simulink model "online_robot_2024b"  (R2024b)
settings: Solver=FixedStepAuto  StartTime=0.0  StopTime=inf  RelTol=1e-3
undefined symbols (not defined in the file): control_par, controller_index, d, D, is_real_robot, k_theta, k_x, k_y, P_INIT_EKF, q_goal_task1, q_goal_task2, q_init, r, R_2, R_5, R_bad, R_good, T_s, Ts, X, Y
libraries: robotlib x6, simulink x5, sharedtransform x1
(part 1 of 2)
settings Model: SimulationMode=accelerator  Creator=dallaliber  LastModifiedBy=HOSAM
settings OptimizationCC: DefaultParameterBehavior=Inlined  EnhancedBackFolding=on  PassReuseOutputArgsAs=Individual arguments  ZeroExternalMemoryAtStartup=off  ZeroInternalMemoryAtStartup=off  MaxStackSize=64  OptimizeBlockOrder=speed  DifferentSizesBufferReuse=on  OptimizationCustomize=off  EfficientTunableParamExpr=on
settings DebuggingCC: ParameterTunabilityLossMsg=error
settings HardwareCC: ProdBitPerPointer=32  ProdBitPerSizeT=32  ProdBitPerPtrDiffT=32  ProdLargestAtomicFloat=None  ProdIntDivRoundTo=Undefined  ProdEndianess=Unspecified  ProdWordSize=32  ProdHWDeviceType=Generic->Unspecified (assume 32-bit Generic)
settings SFSimCC: MATLABDynamicMemAlloc=off
settings RTWCC: Description=Embedded Coder  SystemTargetFile=ert.tlc  HardwareBoard=Robot Operating System (ROS)  TLCOptions="-aInlineSetEventsForThisBaseRateFcn=TLC_FALSE -aSuppressMultiTaskScheduler=TLC_FALSE  -aRateBasedStepFcn=0"  TemplateMakefile=ert_default_tmf  Toolchain=Catkin  TargetLang=C++
settings CodeAppCC: ForceParamTrailComments=on  IgnoreCustomStorageClasses=off  OperatorAnnotations=on  SimulinkDataObjDesc=on  SFDataObjDesc=on  InsertBlockDesc=on
settings ERTTargetCC: DynamicArrayContainerType=coder::array
settings ConfigComp: CovBoundaryAbsTol=1.0e-5

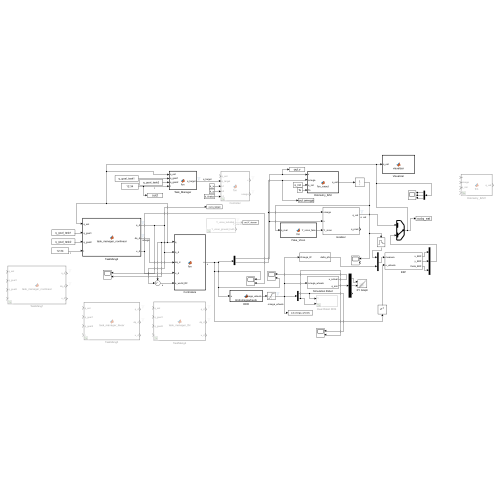
[thumbnail: Simulink's stored preview of the top-level diagram]
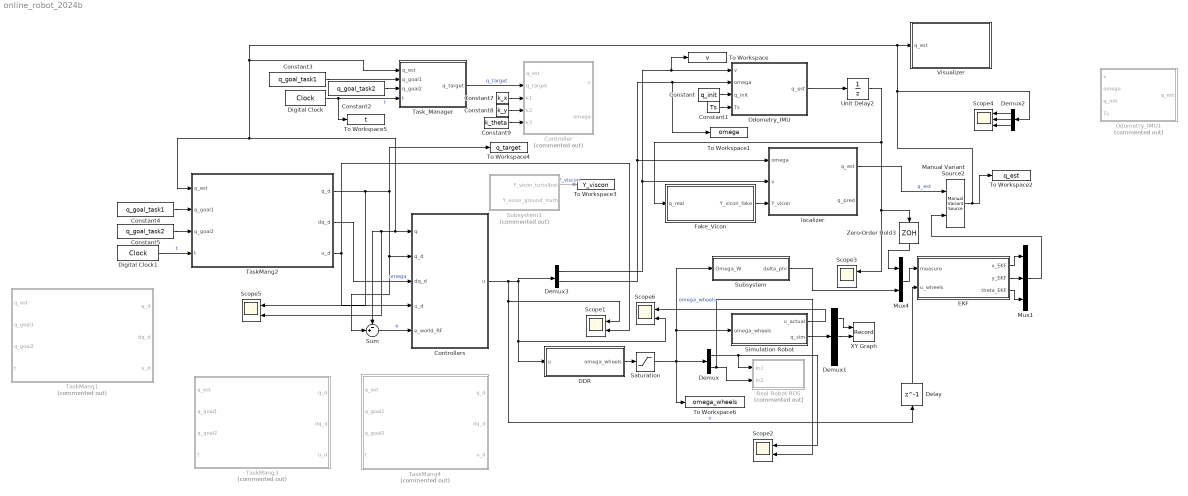
== system online_robot_2024b ==
  Constant : Constant  Value=q_init  SampleTime=Ts
  Constant1 : Constant  Value=Ts  SampleTime=Ts
  Constant2 : Constant  Value=q_goal_task2  SampleTime=Ts
  Constant3 : Constant  Value=q_goal_task1  SampleTime=Ts
  Constant4 : Constant  Value=q_goal_task1  SampleTime=Ts
  Constant5 : Constant  Value=q_goal_task2  SampleTime=Ts
  Constant7 : Constant  Value=k_x  SampleTime=Ts
  Constant8 : Constant  Value=k_y  SampleTime=Ts
  Constant9 : Constant  Value=k_theta  SampleTime=Ts
  Controller : MATLAB Function  Commented=on  TreatAsAtomicUnit=on
  Controllers : MATLAB Function  TreatAsAtomicUnit=on
  DDR : MATLAB Function  TreatAsAtomicUnit=on
  Delay : Delay  DelayLength=1  InitialCondition=[0;0]  SampleTime=Ts
  Demux : Demux  Outputs=2
  Demux1 : Demux  Outputs=3
  Demux2 : Demux  Outputs=3
  Demux3 : Demux  Outputs=2
  Digital Clock : DigitalClock  SampleTime=Ts
  Digital Clock1 : DigitalClock  SampleTime=Ts
  EKF : Subsystem
  Fake_Vicon : MATLAB Function  TreatAsAtomicUnit=on
  Manual Variant Source2 : simulink/Signal Routing/Manual Variant Source  NumChoices=2  LabelModeActiveChoice=V_2
  Mux1 : Mux  Inputs=3
  Mux4 : Mux  Inputs=2
  Odometry_IMU : MATLAB Function  TreatAsAtomicUnit=on
  Odometry_IMU1 : MATLAB Function  Commented=on  TreatAsAtomicUnit=on
  Real Robot ROS : Subsystem  Commented=on
  Saturation : Saturate  UpperLimit=10  LowerLimit=-10
  Scope{1..3,5..6} (5 alike) : Scope  NumInputPorts=2
  Scope4 : Scope  NumInputPorts=3
  Simulation Robot : Subsystem
  Subsystem : Subsystem
  Subsystem1 : Subsystem  Commented=on
  Sum : Sum  Inputs=-+|
  TaskMang1 : MATLAB Function  Commented=on  TreatAsAtomicUnit=on
  TaskMang2 : MATLAB Function  TreatAsAtomicUnit=on
  TaskMang3 : MATLAB Function  Commented=on  TreatAsAtomicUnit=on
  TaskMang4 : MATLAB Function  Commented=on  TreatAsAtomicUnit=on
  Task_Manager : MATLAB Function  TreatAsAtomicUnit=on
  To Workspace : ToWorkspace  VariableName=v  SampleTime=Ts
  To Workspace1 : ToWorkspace  VariableName=omega  SampleTime=Ts
  To Workspace2 : ToWorkspace  VariableName=q_est  SampleTime=Ts
  To Workspace3 : ToWorkspace  VariableName=Y_viscon  SampleTime=Ts
  To Workspace4 : ToWorkspace  VariableName=q_target  SampleTime=Ts
  To Workspace5 : ToWorkspace  VariableName=t  SampleTime=Ts
  To Workspace6 : ToWorkspace  VariableName=omega_wheels  SampleTime=Ts
  Unit Delay2 : UnitDelay  InitialCondition=q_init  SampleTime=Ts  HasFrameUpgradeWarning=on
  Visualizer : MATLAB Function  TreatAsAtomicUnit=on
  XY Graph : Record  FileSettingsInternal="{\"entries\":[{\"content\":{\"excelSettings\":{\"content\":{},\"type\":\"Streamout.ExcelSettings\"},\"parquetSettings\":{\"content\":{},\"type\":\"Streamout.ParquetSettings\"}},\"type\":\"Streamout.FileSettingStorage\",\"uuid\":\"\"}],\"packageUris\":[\"http:\\/\\/schema.mathworks.com\\/mf0\\/streamout_blocks\\/R2020a\"],\"version\":\"1.0\"}"  Layout=[1 1]  SignalsInternal="{\"entries\":[{\"content\":{\"signals\":[{\"content\":{\"blockPath\":[],\"dimensions\":[1],\"domain\":\"\",\"lineColor\":\"#a2142f\",\"plots\":[ 1 ],\"port\":1,\"signalID\":1,\"signalName\":\"Demux1:1\"},\"type\":\"RecordBlkView.Signal\",\"uuid\":\"\"},{\"content\":{\"blockPath\":[],\"dimensions\":[1],\"domain\":\"\",\"lineColor\":\"#139fff\",\"plots\":[ 1 ],\"port\":2,\"signalID\":2,\"signalName\":\"Demux1:2\"},\"type\":\"RecordBlkView.Signal\",\"uuid\":\"\"}]},\"type\":\"RecordBlkView.InputSignals\",\"uuid\":\"\"}],\"packageUris\":[\"http:\\/\\/schema.mathworks.com\\/mf0\\/streamout_blocks\\/R2020a\"],\"version\":\"1.0\"}"  VisualizationBindings="{\"xyplotplugin\":{\"info\":[{\"series\":[{\"bindingParametersList\":[{\"parameter\":\"X-Axis\",\"signalID\":1,\"signalName\":\"Demux1:1\"},{\"parameter\":\"Y-Axis\",\"signalID\":2,\"signalName\":\"Demux1:2\"}],\"seriesID\":0}],\"subplotID\":1}]}}"  CompatibilityTag=XY
  Zero-Order Hold3 : ZeroOrderHold  SampleTime=T_s
  localizer : Subsystem
  wires:
  Constant/1 -> Odometry_IMU/3(q_init)
  Constant1/1 -> Odometry_IMU/4(Ts)
  Constant2/1 -> Task_Manager/3(q_goal2)
  Constant3/1 -> Task_Manager/2(q_goal1)
  Odometry_IMU/1(q_est) -> Unit Delay2/1
  Saturation/1 -> Subsystem/1(Omega_W), Simulation Robot/1(omega_wheels), To Workspace6/1, Demux/1  "omega_wheels"
  DDR/1(omega_wheels) -> Saturation/1
  Demux/1 -> Scope2/1, Real Robot ROS/1(In1)
  Demux/2 -> Scope2/2, Real Robot ROS/2(In2)
  Digital Clock/1 -> To Workspace5/1, Task_Manager/4(t)  "t"
  Subsystem1/1(Y_vicon_turtulbot) -> To Workspace3/1  "Y_viscon"
  Task_Manager/1(q_target) -> Controller/2(q_target)  "q_target"
  Constant7/1 -> Controller/3(k1)
  Constant8/1 -> Controller/4(k2)
  Constant9/1 -> Controller/5(k3)
  Fake_Vicon/1(Y_vicon_fake) -> localizer/3(Y_vicon)
  Unit Delay2/1 -> Zero-Order Hold3/1, Scope3/1, Fake_Vicon/1(q_real)
  Simulation Robot/2(q_sim) -> Demux1/1
  Demux2/3 -> Scope4/3
  Demux2/1 -> Scope4/1
  Demux2/2 -> Scope4/2
  Demux1/1 -> XY Graph/1
  Demux1/2 -> XY Graph/2
  Constant4/1 -> TaskMang2/2(q_goal1)
  Constant5/1 -> TaskMang2/3(q_goal2)
  Digital Clock1/1 -> TaskMang2/4(t)  "t"
  TaskMang2/1(q_d) -> Sum/2, Controllers/2(q_d), To Workspace4/1, Scope5/1
  TaskMang2/2(dq_d) -> Controllers/3(dq_d)  "omega"
  TaskMang2/3(u_d) -> Controllers/4(u_d), Scope1/2
  Sum/1 -> Controllers/5(e_world_RF)  "e"
  Controllers/1(u) -> Delay/1, Scope1/1, Demux3/1, Scope6/2, DDR/1(u)  "u"
  Demux3/1 -> To Workspace/1, Odometry_IMU/1(v), localizer/2(v)
  Demux3/2 -> To Workspace1/1, Odometry_IMU/2(omega), localizer/1(omega)
  EKF/2(y_EKF) -> Mux1/2
  EKF/1(x_EKF) -> Mux1/1
  EKF/3(theta_EKF) -> Mux1/3
  Subsystem/1(delta_phi) -> Mux4/2
  Zero-Order Hold3/1 -> Mux4/1
  Mux4/1 -> EKF/1(measure)
  Manual Variant Source2/1 -> Task_Manager/1(q_est), Controllers/1(q), Scope5/2, Sum/1, TaskMang2/1(q_est), Visualizer/1(q_est), Demux2/1, To Workspace2/1
  localizer/1(q_est) -> Manual Variant Source2/1  "q_est"
  Mux1/1 -> Manual Variant Source2/2
  Simulation Robot/1(u_actual) -> Scope6/1
  Delay/1 -> EKF/2(u_wheels)

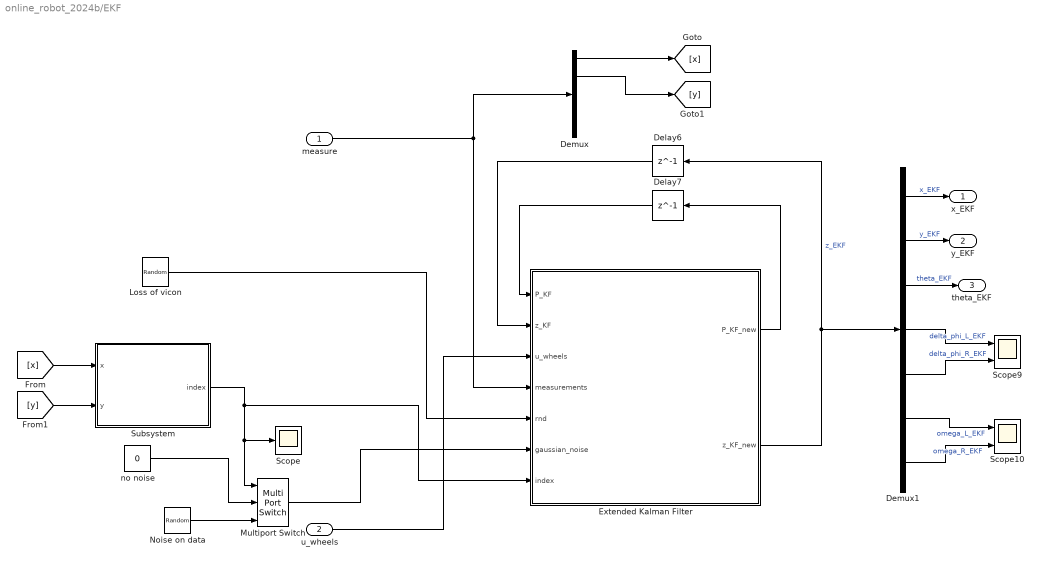
== system online_robot_2024b/EKF ==
  measure : Inport
  u_wheels : Inport  Port=2
  " Loss of vicon" : UniformRandomNumber  Minimum=0  SampleTime=Ts
  Delay6 : Delay  DelayLength=1  InitialCondition=[q_init; 0; 0; 0; 0]  SampleTime=Ts
  Delay7 : Delay  DelayLength=1  InitialCondition=P_INIT_EKF  SampleTime=Ts
  Demux : Demux  Outputs=5
  Demux1 : Demux  Outputs=7
  Extended Kalman Filter : MATLAB Function  TreatAsAtomicUnit=on
  Multiport Switch : MultiPortSwitch  Inputs=2  SaturateOnIntegerOverflow=off  InputSameDT=off
  Noise on data : RandomNumber  Variance=0.02^2  SampleTime=Ts
  Scope : Scope
  Scope10 : Scope  NumInputPorts=2
  Scope9 : Scope  NumInputPorts=2
  Subsystem : Subsystem
  no noise : Constant  Value=0
  x_EKF : Outport
  y_EKF : Outport  Port=2
  theta_EKF : Outport  Port=3
  wires:
  Demux1/6 -> Scope10/1  "omega_L_EKF"
  Demux1/3 -> theta_EKF/1  "theta_EKF"
  Delay6/1 -> Extended Kalman Filter/2(z_KF)
  Delay7/1 -> Extended Kalman Filter/1(P_KF)
  Demux1/5 -> Scope9/2  "delta_phi_R_EKF"
  Demux1/7 -> Scope10/2  "omega_R_EKF"
  Extended Kalman Filter/1(P_KF_new) -> Delay7/1
  Multiport Switch/1 -> Extended Kalman Filter/6(gaussian_noise)
  " Loss of vicon"/1 -> Extended Kalman Filter/5(rnd)
  Demux1/1 -> x_EKF/1  "x_EKF"
  Demux1/4 -> Scope9/1  "delta_phi_L_EKF"
  u_wheels/1 -> Extended Kalman Filter/3(u_wheels)
  Extended Kalman Filter/2(z_KF_new) -> Demux1/1, Delay6/1  "z_EKF"
  measure/1 -> Demux/1, Extended Kalman Filter/4(measurements)
  Demux1/2 -> y_EKF/1  "y_EKF"
  Subsystem/1(index) -> Extended Kalman Filter/7(index), Multiport Switch/1, Scope/1
  [x] -> Subsystem/1(x)
  Noise on data/1 -> Multiport Switch/3
  no noise/1 -> Multiport Switch/2
  [y] -> Subsystem/2(y)
  Demux/1 -> [x]
  Demux/2 -> [y]

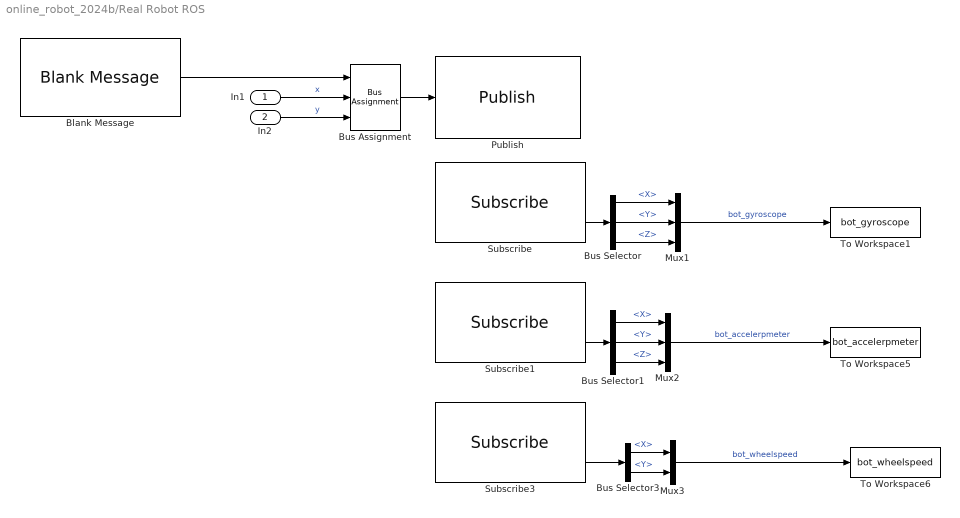
== system online_robot_2024b/Real Robot ROS ==
  In1 : Inport
  In2 : Inport  Port=2
  Blank Message : robotlib/Blank Message  messageClass=Message  entityType=geometry_msgs/Vector3  messageType=geometry_msgs/Vector3  SampleTime=0.04  legacyBusStruct=off
  Bus Assignment : BusAssignment  AssignedSignals=X,Y
  Bus Selector : BusSelector  OutputSignals=X,Y,Z
  Bus Selector1 : BusSelector  OutputSignals=X,Y,Z
  Bus Selector3 : BusSelector  OutputSignals=X,Y
  Mux1 : Mux  Inputs=3
  Mux2 : Mux  Inputs=3
  Mux3 : Mux  Inputs=2
  Publish : robotlib/Publish  topicSource=Select from ROS network  topic=/turtlebot_09/cmd_wheels  messageType=geometry_msgs/Vector3  legacyBusStruct=off  messageQueueLength=1
  Subscribe : robotlib/Subscribe  topicSource=Select from ROS network  topic=/turtlebot_09/gyroscope  messageType=geometry_msgs/Vector3  SampleTime=0.04  legacyBusStruct=off  messageQueueLength=1
  Subscribe1 : robotlib/Subscribe  topicSource=Select from ROS network  topic=/turtlebot_09/accelerometer  messageType=geometry_msgs/Vector3  SampleTime=0.04  legacyBusStruct=off  messageQueueLength=1
  Subscribe3 : robotlib/Subscribe  topicSource=Select from ROS network  topic=/turtlebot_09/wheelSpeeds  messageType=geometry_msgs/Vector3  SampleTime=0.04  legacyBusStruct=off  messageQueueLength=1
  To Workspace1 : ToWorkspace  VariableName=bot_gyroscope  SaveFormat=Timeseries  SampleTime=Ts
  To Workspace5 : ToWorkspace  VariableName=bot_accelerpmeter  SaveFormat=Timeseries  SampleTime=Ts
  To Workspace6 : ToWorkspace  VariableName=bot_wheelspeed  SaveFormat=Timeseries  SampleTime=Ts
  wires:
  Subscribe1/2 -> Bus Selector1/1
  Bus Selector1/1 -> Mux2/1  "<X>"
  Mux2/1 -> To Workspace5/1  "bot_accelerpmeter"
  Bus Assignment/1 -> Publish/1
  Subscribe/2 -> Bus Selector/1
  In2/1 -> Bus Assignment/3  "y"
  Bus Selector/2 -> Mux1/2  "<Y>"
  Bus Selector/1 -> Mux1/1  "<X>"
  Bus Selector3/1 -> Mux3/1  "<X>"
  Bus Selector3/2 -> Mux3/2  "<Y>"
  Bus Selector1/3 -> Mux2/3  "<Z>"
  Bus Selector1/2 -> Mux2/2  "<Y>"
  Mux3/1 -> To Workspace6/1  "bot_wheelspeed"
  Mux1/1 -> To Workspace1/1  "bot_gyroscope"
  Subscribe3/2 -> Bus Selector3/1
  In1/1 -> Bus Assignment/2  "x"
  Blank Message/1 -> Bus Assignment/1
  Bus Selector/3 -> Mux1/3  "<Z>"

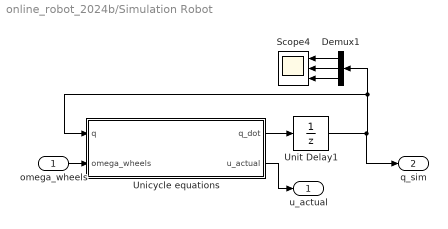
== system online_robot_2024b/Simulation Robot ==
  omega_wheels : Inport
  Demux1 : Demux  Outputs=3
  Scope4 : Scope  NumInputPorts=3
  Unicycle equations : MATLAB Function  TreatAsAtomicUnit=on
  Unit Delay1 : UnitDelay  InitialCondition=q_init  SampleTime=Ts  HasFrameUpgradeWarning=on
  u_actual : Outport
  q_sim : Outport  Port=2
  wires:
  Unicycle equations/1(q_dot) -> Unit Delay1/1
  Demux1/2 -> Scope4/2
  Demux1/1 -> Scope4/1
  Unicycle equations/2(u_actual) -> u_actual/1
  omega_wheels/1 -> Unicycle equations/2(omega_wheels)
  Unit Delay1/1 -> q_sim/1, Unicycle equations/1(q), Demux1/1
  Demux1/3 -> Scope4/3

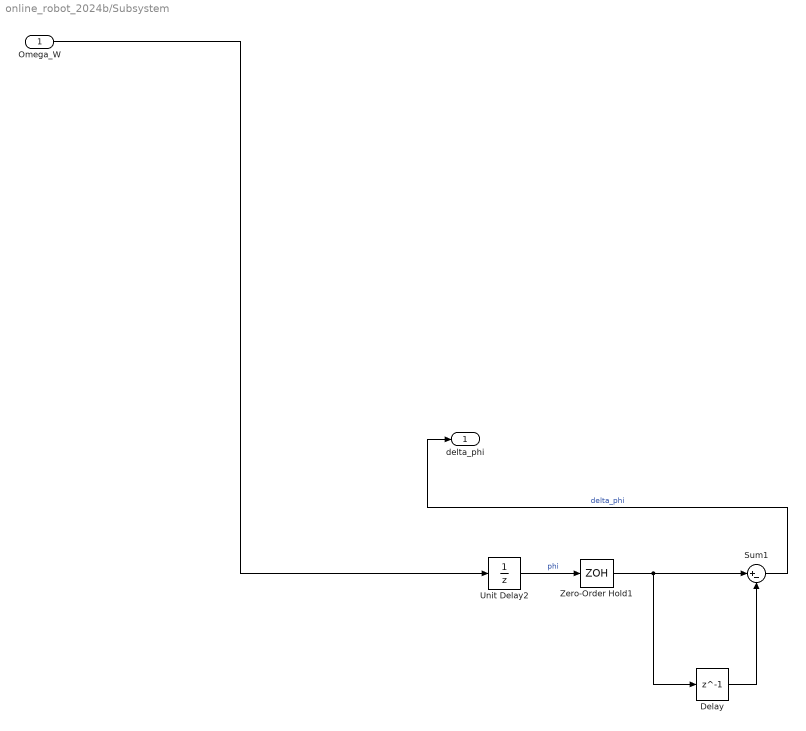
== system online_robot_2024b/Subsystem ==
  Omega_W : Inport
  Delay : Delay  DelayLength=1  InitialCondition=[0;0]  SampleTime=T_s
  Sum1 : Sum  Inputs=|+-
  Unit Delay2 : UnitDelay  InitialCondition=[0;0]  SampleTime=Ts  HasFrameUpgradeWarning=on
  Zero-Order Hold1 : ZeroOrderHold  SampleTime=T_s
  delta_phi : Outport
  wires:
  Sum1/1 -> delta_phi/1  "delta_phi"
  Omega_W/1 -> Unit Delay2/1
  Zero-Order Hold1/1 -> Sum1/1, Delay/1
  Delay/1 -> Sum1/2
  Unit Delay2/1 -> Zero-Order Hold1/1  "phi"

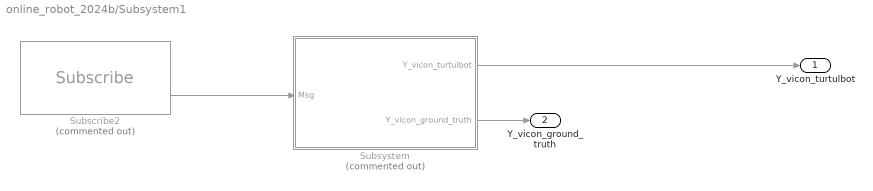
== system online_robot_2024b/Subsystem1 ==
  Subscribe2 : robotlib/Subscribe  Commented=on  topicSource=Select from ROS network  topic=/turtlebot_09/odom  messageType=nav_msgs/Odometry  SampleTime=Ts  legacyBusStruct=off  messageQueueLength=1
      settings: LibrarySourceBlock=roslib/ROS/Subscribe
  Subsystem : Subsystem  Commented=on
  Y_vicon_turtulbot : Outport
  Y_vicon_ground_truth : Outport  Port=2
  wires:
  Subscribe2/2 -> Subsystem/1(Msg)
  Subsystem/2(Y_vicon_ground_truth) -> Y_vicon_ground_truth/1
  Subsystem/1(Y_vicon_turtulbot) -> Y_vicon_turtulbot/1

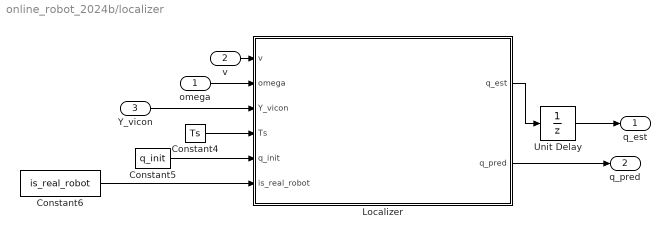
== system online_robot_2024b/localizer ==
  omega : Inport
  v : Inport  Port=2
  Y_vicon : Inport  Port=3
  Constant4 : Constant  Value=Ts
  Constant5 : Constant  Value=q_init
  Constant6 : Constant  Value=is_real_robot
  Localizer : MATLAB Function  TreatAsAtomicUnit=on
  Unit Delay : UnitDelay  InitialCondition=q_init  SampleTime=Ts  HasFrameUpgradeWarning=on
  q_est : Outport
  q_pred : Outport  Port=2
  wires:
  Constant6/1 -> Localizer/6(is_real_robot)
  Y_vicon/1 -> Localizer/3(Y_vicon)
  Localizer/1(q_est) -> Unit Delay/1
  omega/1 -> Localizer/2(omega)
  Constant4/1 -> Localizer/4(Ts)
  Constant5/1 -> Localizer/5(q_init)
  Unit Delay/1 -> q_est/1
  v/1 -> Localizer/1(v)
  Localizer/2(q_pred) -> q_pred/1

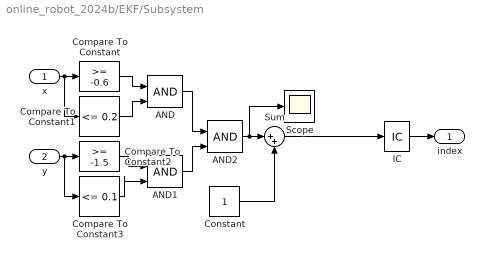
== system online_robot_2024b/EKF/Subsystem ==
  x : Inport
  y : Inport  Port=2
  AND : Logic  IconShape=distinctive  AllPortsSameDT=off  OutDataTypeStr=boolean
  AND1 : Logic  IconShape=distinctive  AllPortsSameDT=off  OutDataTypeStr=boolean
  AND2 : Logic  IconShape=distinctive  AllPortsSameDT=off  OutDataTypeStr=boolean
  Compare To Constant : simulink/Logic and Bit Operations/Compare To Constant  relop=>=  const=-0.6  OutDataTypeStr=boolean
  Compare To Constant1 : simulink/Logic and Bit Operations/Compare To Constant  relop=<=  const=0.2  OutDataTypeStr=boolean
  Compare To Constant2 : simulink/Logic and Bit Operations/Compare To Constant  relop=>=  const=-1.5  OutDataTypeStr=boolean
  Compare To Constant3 : simulink/Logic and Bit Operations/Compare To Constant  relop=<=  const=0.1  OutDataTypeStr=boolean
  Constant : Constant
  IC : InitialCondition
  Scope : Scope
  Sum : Sum  Inputs=|++
  index : Outport
  wires:
  AND/1 -> AND2/1
  x/1 -> Compare To Constant1/1, Compare To Constant/1
  Compare To Constant2/1 -> AND1/1
  Compare To Constant/1 -> AND/1
  AND1/1 -> AND2/2
  Compare To Constant3/1 -> AND1/2
  Compare To Constant1/1 -> AND/2
  y/1 -> Compare To Constant3/1, Compare To Constant2/1
  AND2/1 -> Scope/1, Sum/1
  Constant/1 -> Sum/2
  IC/1 -> index/1
  Sum/1 -> IC/1

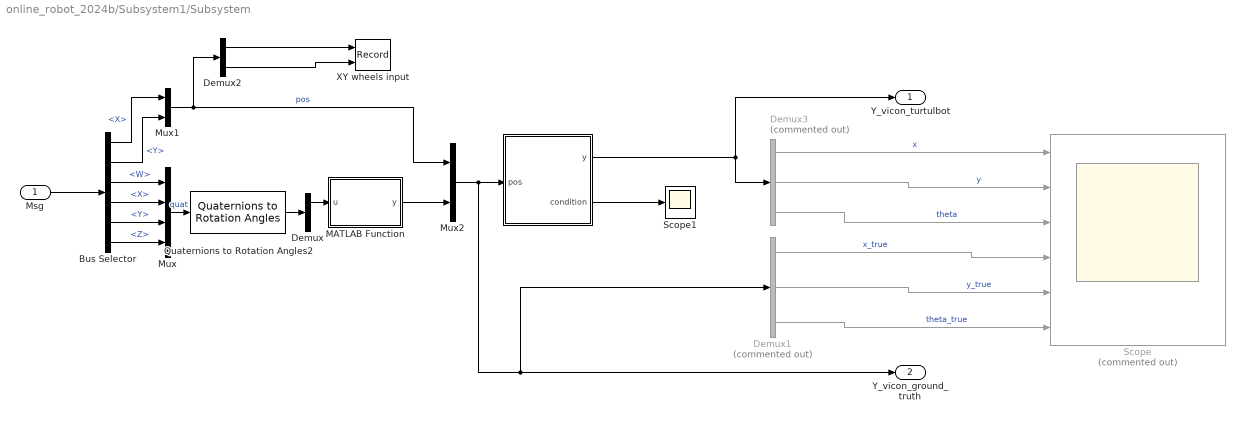
== system online_robot_2024b/Subsystem1/Subsystem ==
  Msg : Inport
  " " : MATLAB Function  TreatAsAtomicUnit=on
  Bus Selector : BusSelector  OutputSignals=Pose.Pose.Position.X,Pose.Pose.Position.Y,Pose.Pose.Orientation.W,Pose.Pose.Orientation.X,Pose.Pose.Orientation.Y,Pose.Pose.Orientation.Z
  Demux : Demux  Outputs=3
  Demux1 : Demux  Commented=on  Outputs=3
  Demux2 : Demux  Outputs=2
  Demux3 : Demux  Commented=on  Outputs=3
  MATLAB Function : MATLAB Function  TreatAsAtomicUnit=on
  Mux : Mux
  Mux1 : Mux  Inputs=2
  Mux2 : Mux  Inputs=2
  Quaternions to Rotation Angles2 : sharedtransform/Quaternions to Rotation Angles  rotationOrder=ZYX  aMode=aMode
  Scope : Scope  Commented=on  NumInputPorts=6
  Scope1 : Scope
  XY wheels input : Record  FileSettingsInternal="{\"entries\":[{\"content\":{\"excelSettings\":{\"content\":{},\"type\":\"Streamout.ExcelSettings\"},\"parquetSettings\":{\"content\":{},\"type\":\"Streamout.ParquetSettings\"}},\"type\":\"Streamout.FileSettingStorage\",\"uuid\":\"\"}],\"packageUris\":[\"http:\\/\\/schema.mathworks.com\\/mf0\\/streamout_blocks\\/R2020a\"],\"version\":\"1.0\"}"  Layout=[1 1]  SignalsInternal="{\"entries\":[{\"content\":{},\"type\":\"RecordBlkView.InputSignals\",\"uuid\":\"\"}],\"packageUris\":[\"http:\\/\\/schema.mathworks.com\\/mf0\\/streamout_blocks\\/R2020a\"],\"version\":\"1.0\"}"  VisualizationBindings="{\"xyplotplugin\":{\"info\":[{\"series\":[],\"subplotID\":1}]}}"  CompatibilityTag=XY
  Y_vicon_turtulbot : Outport
  Y_vicon_ground_truth : Outport  Port=2
  wires:
  Msg/1 -> Bus Selector/1
  Mux2/1 -> Demux1/1, Y_vicon_ground_truth/1, " "/1(pos)
  Bus Selector/3 -> Mux/1  "<W>"
  Mux/1 -> Quaternions to Rotation Angles2/1  "quat"
  Bus Selector/2 -> Mux1/2  "<Y>"
  Demux3/1 -> Scope/1  "x"
  Bus Selector/6 -> Mux/4  "<Z>"
  Bus Selector/1 -> Mux1/1  "<X>"
  " "/1(y) -> Y_vicon_turtulbot/1, Demux3/1
  Demux1/2 -> Scope/5  "y_true"
  Bus Selector/4 -> Mux/2  "<X>"
  Bus Selector/5 -> Mux/3  "<Y>"
  Demux1/3 -> Scope/6  "theta_true"
  " "/2(condition) -> Scope1/1
  Demux3/3 -> Scope/3  "theta"
  Demux3/2 -> Scope/2  "y"
  Demux1/1 -> Scope/4  "x_true"
  MATLAB Function/1(y) -> Mux2/2
  Mux1/1 -> Demux2/1, Mux2/1  "pos"
  Quaternions to Rotation Angles2/1 -> Demux/1
  Demux/1 -> MATLAB Function/1(u)
  Demux2/1 -> XY wheels input/1
  Demux2/2 -> XY wheels input/2

== matlab function online_robot_2024b/Simulation Robot/Unicycle equations ==
  data: q input; omega_wheels input; q_dot output; r parameter; d parameter; u_actual output
function [q_dot, u_actual] = q_dot(q, omega_wheels, r, d)
u_actual = [r/2, r/2;-r/d, r/d]*omega_wheels;
theta = q(3);
q_dot = [[cos(theta), 0];[sin(theta), 0];[0,1]]*u_actual;

== matlab function online_robot_2024b/Task_Manager ==
  data: q_est input; q_target output; q_goal1 input; q_goal2 input; t input
function q_target = fcn(q_est, q_goal1, q_goal2, t)
    coder.extrinsic('disp');    

    % Default initialization to avoid Simulink Coder errors
    q_target = q_goal1; 
    
    % Define persistent variables to store state and timing information
    persistent state t_reached
    if isempty(state)
        state = 1; % Robot starts from Task 1
        t_reached = 0; % Stores the time when each target is reached
    end

    % --- Intermediate Waypoints for Collision-Free Navigation ---
    q_wp1 = [-0.20; -1.10; 0];    % First waypoint: pass below the gray obstacle
    q_wp2 = [-0.20; -0.30; pi/2]; % Second waypoint: rotate upward toward the corridor
    q_wp3 = [1.45; -0.30; 0];     % Third waypoint: exit corridor and prepare for Task 3
    
    % --- Starting Point of Task 3 (Circle Path) ---
    q_start_task3 = [2.00; -0.60; 0]; % Positioned below the brown obstacle for circle alignment

    % --- Task 3 Parameters (Circular Motion) ---
    R_circle = 0.60;      % Circle radius chosen for safe obstacle avoidance
    omega_circle = 0.35;  % Angular speed kept low to reduce Kalman filter drift

    % --- Euclidean Distance Calculations ---
    dist1 = sqrt((q_est(1)-q_goal1(1))^2 + (q_est(2)-q_goal1(2))^2);
    dist_wp1 = sqrt((q_est(1)-q_wp1(1))^2 + (q_est(2)-q_wp1(2))^2);
    dist_wp2 = sqrt((q_est(1)-q_wp2(1))^2 + (q_est(2)-q_wp2(2))^2);
    dist2 = sqrt((q_est(1)-q_goal2(1))^2 + (q_est(2)-q_goal2(2))^2);
    dist_wp3 = sqrt((q_est(1)-q_wp3(1))^2 + (q_est(2)-q_wp3(2))^2);
    dist_start3 = sqrt((q_est(1)-q_start_task3(1))^2 + (q_est(2)-q_start_task3(2))^2);

    % --- Target Reaching Thresholds ---
    thresh_strict = 0.05; % Strict threshold for final targets
    thresh_loose = 0.15;  % Looser threshold for smooth waypoint transitions

    % --- State Machine Logic ---
    switch state
        
        case 1 % Move toward Task 1
            q_target = q_goal1;

            if dist1 < thresh_strict
                state = 2; 
                t_reached = t; % Save arrival time for timer
                fprintf('Goal 1 Reached\n');
            end
            
        case 2 % Wait 1 second at Task 1
            q_target = q_goal1;

            if (t - t_reached) >= 1.0
                state = 3;
                fprintf('Moving to Waypoint 1\n');
            end
            
        case 3 % Move toward Waypoint 1
            q_target = q_wp1;

            if dist_wp1 < thresh_loose
                state = 4;
                fprintf('Waypoint 1 Cleared\n');
            end
            
        case 4 % Move toward Waypoint 2
            q_target = q_wp2;

            if dist_wp2 < thresh_loose
                state = 5;
                fprintf('Waypoint 2 Cleared\n');
            end
            
        case 5 % Move toward Task 2
            q_target = q_goal2;

            if dist2 < thresh_strict
                state = 6; 
                fprintf('Goal 2 Reached\n');
            end
            
        case 6 % Move toward Waypoint 3 before starting circle motion
            q_target = q_wp3;

            if dist_wp3 < thresh_loose
                state = 7;
                fprintf('Waypoint 3 Cleared\n');
            end
            
        case 7 % Move toward Task 3 starting point
            q_target = q_start_task3;

            if dist_start3 < thresh_strict
                state = 8; 
                t_reached = t; % Save arrival time for Task 3 timer
                fprintf('Task 3 Start Point Reached\n');
            end
            
        case 8 % Wait 1 second before starting circular motion
            q_target = q_start_task3;

            if (t - t_reached) >= 1.0
                state = 9; 
                t_reached = t; % Reset timer for circular trajectory
                fprintf('Starting Circle\n');
            end
            
        case 9 % Task 3: Follow circular trajectory around brown obstacle
            
            % Virtual rabbit technique:
            % Move the target slightly ahead to prevent spinning in place
            look_ahead = 0.4;
            elapsed = (t - t_reached) + look_ahead;
            
            % Stop after approximately 1.5 revolutions
            if elapsed > 28
                elapsed = 28; 
            end
            
            % Shifted circle equation to ensure smooth tangent entry
            x_d = q_start_task3(1) + R_circle * sin(omega_circle * elapsed);
            y_d = q_start_task3(2) + R_circle * (1 - cos(omega_circle * elapsed));

            % Continuous orientation update
            theta_d = wrapToPi(omega_circle * elapsed);
            
            q_target = [x_d; y_d; theta_d];
            
        otherwise % Default fallback state to prevent Simulink crash
            q_target = q_goal1;
    end
end

== matlab function online_robot_2024b/TaskMang1 ==
  data: q_est input; q_d output; q_goal1 input; dq_d output; q_goal2 input; t input; u_d output
function [q_d, dq_d, u_d] = task_manager_nonlinear(q_est, q_goal1, q_goal2, t)
%TASK_MANAGER_NONLINEAR
% State-machine task manager for the nonlinear trajectory tracking controller.

persistent state t_reached theta_hold

if isempty(state)
    state = 1;
    t_reached = 0;
    theta_hold = q_est(3);
end

%% Parameters
v_ref = 0.18;
v_min = 0.035;
lookahead = 0.50;

wp_tol = 0.15;
goal_tol = 0.07;

k_theta = 1.5;
omega_max = 1.4;

%% Waypoints
q_wp1 = [-0.20; -1.10; 0.0];
q_wp2 = [-0.20; -0.30; pi/2];
q_wp3 = [1.45; -0.30; 0.0];

q_start_task3 = [2.00; -0.60; 0.0];

%% Circle parameters
R_circle = 0.60;
omega_circle = 0.35;
look_ahead_time = 0.45;
circle_duration = 28.0;

%% Select target
target = q_goal1;
mode = 0;

switch state
    case 1
        target = q_goal1;
        if pos_dist(q_est, q_goal1) < goal_tol
            state = 2;
            t_reached = t;
            theta_hold = q_goal1(3);
        end

    case 2
        target = q_goal1;
        mode = 2;
        if (t - t_reached) >= 1.0
            state = 3;
        end

    case 3
        target = q_wp1;
        if pos_dist(q_est, q_wp1) < wp_tol
            state = 4;
        end

    case 4
        target = q_wp2;
        if pos_dist(q_est, q_wp2) < wp_tol
            state = 5;
        end

    case 5
        target = q_goal2;
        if pos_dist(q_est, q_goal2) < goal_tol
            state = 6;
            t_reached = t;
        end

    case 6
        target = q_wp3;
        if pos_dist(q_est, q_wp3) < wp_tol
            state = 7;
        end

    case 7
        target = q_start_task3;
        if pos_dist(q_est, q_start_task3) < goal_tol
            state = 8;
            t_reached = t;
            theta_hold = q_start_task3(3);
        end

    case 8
        target = q_start_task3;
        mode = 2;
        if (t - t_reached) >= 1.0
            state = 9;
            t_reached = t;
        end

    case 9
        mode = 1;

    otherwise
        target = q_goal1;
end

%% Generate reference
if mode == 1
    elapsed = (t - t_reached) + look_ahead_time;
    elapsed = min(elapsed, circle_duration);

    x_d = q_start_task3(1) + R_circle*sin(omega_circle*elapsed);
    y_d = q_start_task3(2) + R_circle*(1 - cos(omega_circle*elapsed));

    dx_d = R_circle*omega_circle*cos(omega_circle*elapsed);
    dy_d = R_circle*omega_circle*sin(omega_circle*elapsed);

    theta_d = atan2(dy_d, dx_d);
    v_d = sqrt(dx_d^2 + dy_d^2);
    omega_d = omega_circle;

    q_d = [x_d; y_d; theta_d];
    dq_d = [dx_d; dy_d; omega_d];
    u_d = [v_d; omega_d];

elseif mode == 2
    q_d = [target(1); target(2); theta_hold];
    dq_d = [0; 0; 0];
    u_d = [0; 0];

else
    dx = target(1) - q_est(1);
    dy = target(2) - q_est(2);
    dist = hypot(dx, dy);

    theta_d = atan2(dy, dx);
    theta_err = wrap_pi(theta_d - q_est(3));

    speed_scale_dist = min(1.0, dist/lookahead);
    speed_scale_heading = max(0.20, cos(theta_err));

    v_d = v_ref * speed_scale_dist * speed_scale_heading;

    if dist > goal_tol
        v_d = max(v_d, v_min);
    else
        v_d = 0;
    end

    omega_d = k_theta * theta_err;
    omega_d = saturate(omega_d, omega_max);

    q_d = [target(1); target(2); theta_d];
    dq_d = [v_d*cos(theta_d); v_d*sin(theta_d); omega_d];
    u_d = [max(v_d, 1e-3); omega_d];

    if dist < goal_tol
        q_d = [target(1); target(2); target(3)];
        dq_d = [0; 0; 0];
        u_d = [0; 0];
    end
end

end

function d = pos_dist(q, p)
d = hypot(q(1)-p(1), q(2)-p(2));
end

function a = wrap_pi(a)
a = atan2(sin(a), cos(a));
end

function y = saturate(x, lim)
y = max(min(x, lim), -lim);
end

== matlab function online_robot_2024b/TaskMang2 ==
  settings: updateMethod=DISCRETE  sampleTime=Ts
  data: q_est input; q_d output; q_goal1 input; dq_d output; q_goal2 input; t input; u_d output
function [q_d, dq_d, u_d] = task_manager_nonlinear(q_est, q_goal1, q_goal2, t)
%TASK_MANAGER_NONLINEAR
% State-machine task manager for the nonlinear trajectory tracking controller.

persistent state t_reached theta_hold

if isempty(state)
    state = 1;
    t_reached = 0;
    theta_hold = q_est(3);
end

%% Parameters
v_ref = 0.18;
v_min = 0.035;
lookahead = 0.50;

wp_tol = 0.15;
goal_tol = 0.07;

k_theta = 1.5;
omega_max = 1.4;

%% Waypoints
q_wp1 = [-0.20; -1.10; 0.0];
q_wp2 = [-0.20; -0.30; pi/2];
q_wp3 = [1.45; -0.30; 0.0];

q_start_task3 = [2.00; -0.60; 0.0];

%% Circle parameters
R_circle = 0.60;
omega_circle = 0.35;
look_ahead_time = 0.45;
circle_duration = 28.0;

%% Select target
target = q_goal1;
mode = 0;

switch state
    case 1
        target = q_goal1;
        if pos_dist(q_est, q_goal1) < goal_tol
            state = 2;
            t_reached = t;
            theta_hold = q_goal1(3);
        end

    case 2
        target = q_goal1;
        mode = 2;
        if (t - t_reached) >= 1.0
            state = 3;
        end

    case 3
        target = q_wp1;
        if pos_dist(q_est, q_wp1) < wp_tol
            state = 4;
        end

    case 4
        target = q_wp2;
        if pos_dist(q_est, q_wp2) < wp_tol
            state = 5;
        end

    case 5
        target = q_goal2;
        if pos_dist(q_est, q_goal2) < goal_tol
            state = 6;
            t_reached = t;
        end

    case 6
        target = q_wp3;
        if pos_dist(q_est, q_wp3) < wp_tol
            state = 7;
        end

    case 7
        target = q_start_task3;
        if pos_dist(q_est, q_start_task3) < goal_tol
            state = 8;
            t_reached = t;
            theta_hold = q_start_task3(3);
        end

    case 8
        target = q_start_task3;
        mode = 2;
        if (t - t_reached) >= 1.0
            state = 9;
            t_reached = t;
        end

    case 9
        mode = 1;

    otherwise
        target = q_goal1;
end

%% Generate reference
if mode == 1
    elapsed = (t - t_reached) + look_ahead_time;
    elapsed = min(elapsed, circle_duration);

    x_d = q_start_task3(1) + R_circle*sin(omega_circle*elapsed);
    y_d = q_start_task3(2) + R_circle*(1 - cos(omega_circle*elapsed));

    dx_d = R_circle*omega_circle*cos(omega_circle*elapsed);
    dy_d = R_circle*omega_circle*sin(omega_circle*elapsed);

    theta_d = atan2(dy_d, dx_d);
    v_d = sqrt(dx_d^2 + dy_d^2);
    omega_d = omega_circle;

    q_d = [x_d; y_d; theta_d];
    dq_d = [dx_d; dy_d; omega_d];
    u_d = [v_d; omega_d];

elseif mode == 2
    q_d = [target(1); target(2); theta_hold];
    dq_d = [0; 0; 0];
    u_d = [0; 0];

else
    dx = target(1) - q_est(1);
    dy = target(2) - q_est(2);
    dist = hypot(dx, dy);

    theta_d = atan2(dy, dx);
    theta_err = wrap_pi(theta_d - q_est(3));

    speed_scale_dist = min(1.0, dist/lookahead);
    speed_scale_heading = max(0.20, cos(theta_err));

    v_d = v_ref * speed_scale_dist * speed_scale_heading;

    if dist > goal_tol
        v_d = max(v_d, v_min);
    else
        v_d = 0;
    end

    omega_d = k_theta * theta_err;
    omega_d = saturate(omega_d, omega_max);

    q_d = [target(1); target(2); theta_d];
    dq_d = [v_d*cos(theta_d); v_d*sin(theta_d); omega_d];
    u_d = [max(v_d, 1e-3); omega_d];

    if dist < goal_tol
        q_d = [target(1); target(2); target(3)];
        dq_d = [0; 0; 0];
        u_d = [0; 0];
    end
end

end

function d = pos_dist(q, p)
d = hypot(q(1)-p(1), q(2)-p(2));
end

function a = wrap_pi(a)
a = atan2(sin(a), cos(a));
end

function y = saturate(x, lim)
y = max(min(x, lim), -lim);
end

== matlab function online_robot_2024b/TaskMang3 ==
  data: q_est input; q_d output; q_goal1 input; dq_d output; q_goal2 input; t input; u_d output
function [q_d, dq_d, u_d] = task_manager_linear(q_est, q_goal1, q_goal2, t)
%TASK_MANAGER_LINEAR
% State-machine task manager for the linear trajectory tracking controller.
%
% Outputs:
%   q_d  = desired pose [x_d; y_d; theta_d]
%   dq_d = desired inertial velocity [dx_d; dy_d; dtheta_d]
%   u_d  = desired unicycle input [v_d; omega_d]

persistent state t_reached theta_hold

if isempty(state)
    state = 1;
    t_reached = 0;
    theta_hold = q_est(3);
end

%% Parameters
v_ref = 0.16;
v_min = 0.04;
lookahead = 0.45;

wp_tol = 0.14;
goal_tol = 0.06;

k_theta = 1.2;
omega_max = 1.2;

%% Waypoints
q_wp1 = [-0.20; -1.10; 0.0];
q_wp2 = [-0.20; -0.30; pi/2];
q_wp3 = [1.45; -0.30; 0.0];

q_start_task3 = [2.00; -0.60; 0.0];

%% Circle parameters
R_circle = 0.60;
omega_circle = 0.35;
look_ahead_time = 0.4;
circle_duration = 28.0;

%% State machine target selection
target = q_goal1;
mode = 0;  % 0 point target, 1 circle, 2 hold

switch state
    case 1
        target = q_goal1;
        if pos_dist(q_est, q_goal1) < goal_tol
            state = 2;
            t_reached = t;
            theta_hold = q_goal1(3);
        end

    case 2
        target = q_goal1;
        mode = 2;
        if (t - t_reached) >= 1.0
            state = 3;
        end

    case 3
        target = q_wp1;
        if pos_dist(q_est, q_wp1) < wp_tol
            state = 4;
        end

    case 4
        target = q_wp2;
        if pos_dist(q_est, q_wp2) < wp_tol
            state = 5;
        end

    case 5
        target = q_goal2;
        if pos_dist(q_est, q_goal2) < goal_tol
            state = 6;
            t_reached = t;
        end

    case 6
        target = q_wp3;
        if pos_dist(q_est, q_wp3) < wp_tol
            state = 7;
        end

    case 7
        target = q_start_task3;
        if pos_dist(q_est, q_start_task3) < goal_tol
            state = 8;
            t_reached = t;
            theta_hold = q_start_task3(3);
        end

    case 8
        target = q_start_task3;
        mode = 2;
        if (t - t_reached) >= 1.0
            state = 9;
            t_reached = t;
        end

    case 9
        mode = 1;

    otherwise
        target = q_goal1;
end

%% Generate reference
if mode == 1
    elapsed = (t - t_reached) + look_ahead_time;
    elapsed = min(elapsed, circle_duration);

    x_d = q_start_task3(1) + R_circle*sin(omega_circle*elapsed);
    y_d = q_start_task3(2) + R_circle*(1 - cos(omega_circle*elapsed));

    dx_d = R_circle*omega_circle*cos(omega_circle*elapsed);
    dy_d = R_circle*omega_circle*sin(omega_circle*elapsed);

    theta_d = atan2(dy_d, dx_d);
    v_d = sqrt(dx_d^2 + dy_d^2);
    omega_d = omega_circle;

    q_d = [x_d; y_d; theta_d];
    dq_d = [dx_d; dy_d; omega_d];
    u_d = [v_d; omega_d];

elseif mode == 2
    q_d = [target(1); target(2); theta_hold];
    dq_d = [0; 0; 0];
    u_d = [0; 0];

else
    dx = target(1) - q_est(1);
    dy = target(2) - q_est(2);
    dist = hypot(dx, dy);

    theta_d = atan2(dy, dx);
    theta_err = wrap_pi(theta_d - q_est(3));

    speed_scale_dist = min(1.0, dist/lookahead);
    speed_scale_heading = max(0.25, cos(theta_err));

    v_d = v_ref * speed_scale_dist * speed_scale_heading;

    if dist > goal_tol
        v_d = max(v_d, v_min);
    else
        v_d = 0;
    end

    omega_d = k_theta * theta_err;
    omega_d = saturate(omega_d, omega_max);

    q_d = [target(1); target(2); theta_d];
    dq_d = [v_d*cos(theta_d); v_d*sin(theta_d); omega_d];
    u_d = [max(v_d, 1e-3); omega_d];

    if dist < goal_tol
        q_d = [target(1); target(2); target(3)];
        dq_d = [0; 0; 0];
        u_d = [0; 0];
    end
end

end

function d = pos_dist(q, p)
d = hypot(q(1)-p(1), q(2)-p(2));
end

function a = wrap_pi(a)
a = atan2(sin(a), cos(a));
end

function y = saturate(x, lim)
y = max(min(x, lim), -lim);
end

== matlab function online_robot_2024b/Controllers ==
  settings: updateMethod=DISCRETE  sampleTime=Ts
  data: q input; q_d input; dq_d input; u_d input; u output; e_world_RF input; controller_index parameter; control_par parameter
function u = fcn(q, q_d, dq_d, u_d, e_world_RF, controller_index, control_par)
% compute the error in the unicycle RF
    e = zeros(3,1);
    e(1) = cos(q(3))*e_world_RF(1) + sin(q(3))*e_world_RF(2);
    e(2) = -sin(q(3))*e_world_RF(1) + cos(q(3))*e_world_RF(2);
    % e(3) = e_world_RF(3);
    e(3) = atan2(sin(e_world_RF(3)),...
             cos(e_world_RF(3)));
    u_ff = zeros(2,1);
    u_k = zeros(2,1);
    u = zeros(2,1);

    %FBL
    pbd_dot = zeros(2,1);
    pbd_dot(1) = dq_d(1) - control_par(3)*sin(q_d(3))*dq_d(3);
    pbd_dot(2) = dq_d(1) + control_par(3)*cos(q_d(3))*dq_d(3);
    xbd = q_d(1)+control_par(3)*cos(q_d(3));
    ybd = q_d(2)+control_par(3)*sin(q_d(3));
    xb = q(1)+control_par(3)*cos(q(3)); 
    yb = q(2)+control_par(3)*sin(q(3));

    e_tilde = zeros(2,1);
    e_tilde(1) = xbd -xb;
    e_tilde(2) = ybd - yb;


    

    
if controller_index == 1
    % linear controller
    k1 = 2*control_par(2)*control_par(1);
    v_safe = max(abs(u_d(1)), 1e-3);
    k2 = (control_par(2)^2 - u_d(2)^2) / v_safe;
    k3 = k1;
      
    u_ff(1)=u_d(1)*cos(e(3));
    u_ff(2)=u_d(2);
   
    u_k(1)=-e(1)*k1;

   if abs(e(3)) < 1e-6
        sinc_e = 1;
   else
        sinc_e = sin(e(3))/e(3);
   end
    
    u_k(2) = -k2*(u_d(1)*sinc_e)*e(2) - k3*e(3);
    u(1)=u_ff(1) - u_k(1);
    u(2)=u_ff(2) - u_k(2);
   
elseif controller_index == 2
    % nonlinear controller
    u_d(1) = max(u_d(1),1e-3);
    a = sqrt(u_d(1)*control_par(2) + u_d(2)^2);
    k1 = 2*a*control_par(1);
    k2 = control_par(2);
    k3 = k1;
    % feedforward
    u_ff(1)=u_d(1)*cos(e(3));
    u_ff(2)=u_d(2);

    u_k(1)=-k1*e(1);
    if abs(e(3)) < 1e-6
        sinc_e = 1;
    else
        sinc_e = sin(e(3))/e(3);
    end
    
    u_k(2) = -k2*(u_d(1)*sinc_e)*e(2) - k3*e(3);

    u(1)=u_ff(1) - u_k(1);
    u(2)=u_ff(2) - u_k(2);
    
elseif controller_index == 3
    % feedback linearization
    k1 = control_par(1);
    k2 = control_par(2);
    b = control_par(3);
    K = diag([k1,k2]);
    % u_k = [cos(q(3)), sin(q(3));...
    %     -sin(q(3))/b, cos(q(3))/b]*[pbd_dot(1)+k1*(xbd -xb); pbd_dot(2)+k2*(ybd -yb)];
    T = [cos(q(3)), -b*sin(q(3)); sin(q(3)), b*cos(q(3))];
    temp = (pbd_dot+K*e_tilde);

    u = T\temp;
    
else
    u = u_d;
end
if norm(q_d(1:2) - q(1:2)) < 0.001 && norm(u_d) < 1e-6
    u = [0; 0];
end

%% Saturation
v_max = 0.35;
w_max = 2.0;
u(1) = max(min(u(1), v_max), -v_max);
u(2) = max(min(u(2), w_max), -w_max);
end

== matlab function online_robot_2024b/TaskMang4 ==
  data: q_est input; q_d output; q_goal1 input; dq_d output; q_goal2 input; t input; u_d output
function [q_d, dq_d, u_d] = task_manager_fbl(q_est, q_goal1, q_goal2, t)
%TASK_MANAGER_FBL
% State-machine task manager for feedback-linearization controller.
%
% Designed to provide smooth Cartesian reference and velocity.

persistent state t_reached theta_hold last_qd last_t

if isempty(state)
    state = 1;
    t_reached = 0;
    theta_hold = q_est(3);
    last_qd = q_est;
    last_t = t;
end

%% Parameters
v_ref = 0.15;
v_min = 0.03;
lookahead = 0.55;

wp_tol = 0.15;
goal_tol = 0.07;

k_theta = 1.0;
omega_max = 1.2;

%% Waypoints
q_wp1 = [-0.20; -1.10; 0.0];
q_wp2 = [-0.20; -0.30; pi/2];
q_wp3 = [1.45; -0.30; 0.0];

q_start_task3 = [2.00; -0.60; 0.0];

%% Circle parameters
R_circle = 0.60;
omega_circle = 0.30;
look_ahead_time = 0.5;
circle_duration = 31.5;

%% Select target
target = q_goal1;
mode = 0;

switch state
    case 1
        target = q_goal1;
        if pos_dist(q_est, q_goal1) < goal_tol
            state = 2;
            t_reached = t;
            theta_hold = q_goal1(3);
        end

    case 2
        target = q_goal1;
        mode = 2;
        if (t - t_reached) >= 1.0
            state = 3;
        end

    case 3
        target = q_wp1;
        if pos_dist(q_est, q_wp1) < wp_tol
            state = 4;
        end

    case 4
        target = q_wp2;
        if pos_dist(q_est, q_wp2) < wp_tol
            state = 5;
        end

    case 5
        target = q_goal2;
        if pos_dist(q_est, q_goal2) < goal_tol
            state = 6;
            t_reached = t;
        end

    case 6
        target = q_wp3;
        if pos_dist(q_est, q_wp3) < wp_tol
            state = 7;
        end

    case 7
        target = q_start_task3;
        if pos_dist(q_est, q_start_task3) < goal_tol
            state = 8;
            t_reached = t;
            theta_hold = q_start_task3(3);
        end

    case 8
        target = q_start_task3;
        mode = 2;
        if (t - t_reached) >= 1.0
            state = 9;
            t_reached = t;
        end

    case 9
        mode = 1;

    otherwise
        target = q_goal1;
end

%% Generate desired pose and velocity
if mode == 1
    elapsed = (t - t_reached) + look_ahead_time;
    elapsed = min(elapsed, circle_duration);

    x_d = q_start_task3(1) + R_circle*sin(omega_circle*elapsed);
    y_d = q_start_task3(2) + R_circle*(1 - cos(omega_circle*elapsed));

    dx_d = R_circle*omega_circle*cos(omega_circle*elapsed);
    dy_d = R_circle*omega_circle*sin(omega_circle*elapsed);

    theta_d = atan2(dy_d, dx_d);
    v_d = sqrt(dx_d^2 + dy_d^2);
    omega_d = omega_circle;

    q_d = [x_d; y_d; theta_d];
    dq_d = [dx_d; dy_d; omega_d];
    u_d = [v_d; omega_d];

elseif mode == 2
    q_d = [target(1); target(2); theta_hold];
    dq_d = [0; 0; 0];
    u_d = [0; 0];

else
    dx = target(1) - q_est(1);
    dy = target(2) - q_est(2);
    dist = hypot(dx, dy);

    theta_d = atan2(dy, dx);
    theta_err = wrap_pi(theta_d - q_est(3));

    speed_scale_dist = min(1.0, dist/lookahead);
    speed_scale_heading = max(0.25, cos(theta_err));

    v_d = v_ref * speed_scale_dist * speed_scale_heading;

    if dist > goal_tol
        v_d = max(v_d, v_min);
    else
        v_d = 0;
    end

    omega_d = k_theta * theta_err;
    omega_d = saturate(omega_d, omega_max);

    q_d = [target(1); target(2); theta_d];
    dq_d = [v_d*cos(theta_d); v_d*sin(theta_d); omega_d];
    u_d = [v_d; omega_d];

    if dist < goal_tol
        q_d = [target(1); target(2); target(3)];
        dq_d = [0; 0; 0];
        u_d = [0; 0];
    end
end

%% Optional numerical smoothing of dq_d for FBL
dt = t - last_t;

if dt > 1e-6
    dq_num = (q_d - last_qd) / dt;
    dq_num(3) = wrap_pi(q_d(3) - last_qd(3)) / dt;

    alpha = 0.4;
    dq_d = alpha*dq_d + (1-alpha)*dq_num;
end

last_qd = q_d;
last_t = t;

end

function d = pos_dist(q, p)
d = hypot(q(1)-p(1), q(2)-p(2));
end

function a = wrap_pi(a)
a = atan2(sin(a), cos(a));
end

function y = saturate(x, lim)
y = max(min(x, lim), -lim);
end

== matlab function online_robot_2024b/EKF/Extended Kalman Filter ==
  settings: updateMethod=DISCRETE  sampleTime=Ts
  data: P_KF input; P_KF_new output; z_KF input; u_wheels input; measurements input; D parameter; R_5 parameter; r parameter; d parameter; rnd input; gaussian_noise input; z_KF_new output; T_s parameter; index input; R_2 parameter; R_bad parameter; R_good parameter
function [P_KF_new, z_KF_new] = Extended_Kalman_Filter1(P_KF, z_KF, u_wheels, measurements, D, R_5,r, d, rnd, gaussian_noise, T_s,index, R_2,R_bad, R_good)

% z_KF = [x_EKF, y_EKF, theta_EKF, delta_phi_L_EKF, delta_phi_R_EKF, omega_L_EKF, omega_R_EKF]

v_k = r * (z_KF(6) + z_KF(7))/2;
w_k = r * (z_KF(7) - z_KF(6))/d;

theta_mean = z_KF(3) + (w_k * T_s)/2;

F_k = [1, 0, -T_s * v_k * sin(theta_mean), 0, 0, T_s * r * cos(theta_mean)/2 + (T_s)^2 * r * v_k * sin(theta_mean)/(2*d), T_s * r * cos(theta_mean)/2 - (T_s)^2 * r * v_k * sin(theta_mean)/(2*d);
    0, 1, T_s * v_k * cos(theta_mean), 0, 0, T_s * r * sin(theta_mean)/2 - (T_s)^2 * r * v_k * cos(theta_mean)/(2*d), T_s * r * sin(theta_mean)/2 + (T_s)^2 * r * v_k * cos(theta_mean)/(2*d);
    0, 0, 1, 0, 0, (-T_s*r)/d, (T_s*r)/d;
    0, 0, 0, 1, 0, T_s, 0;
    0, 0, 0, 0, 1, 0, T_s;
    0, 0, 0, 0, 0, 1, 0;
    0, 0, 0, 0, 0, 0, 1];

%% Prediction part
% theta_mid = z_KF(3) + 0.5*w_k*T_s;

% z_pred = [
%     z_KF(1) + T_s*v_k*cos(theta_mid);
%     z_KF(2) + T_s*v_k*sin(theta_mid);
%     z_KF(3) + T_s*w_k;
%     z_KF(4) + T_s*z_KF(6);
%     z_KF(5) + T_s*z_KF(7);
%     u_wheels(1);
%     u_wheels(2)
% ];

z_pred = [z_KF(1)+(T_s*r*(z_KF(6)+z_KF(7))/2)*cos(theta_mean + (T_s*r*(z_KF(6)+z_KF(7)))/(2*d));
    z_KF(2)+(T_s*r*(z_KF(6)+z_KF(7))/2)*sin(theta_mean + (T_s*r*(z_KF(7)-z_KF(6)))/(2*d));
    theta_mean + (T_s*r*(z_KF(7)-z_KF(6))/(2*d));
    z_KF(4) + u_wheels(1);
    z_KF(5) + u_wheels(2);
    u_wheels(1);
    u_wheels(2)];

P_pred = F_k * P_KF * F_k' + D;


%% Update

% initialize dimensions
y_measurement = zeros(6,1);
H = zeros(5,7);
R = R_5;  % initialize with largest

m = 0; % actual measurement dimension
if index == 2
    % Robot is INSIDE the zone: High chance of total signal loss
    prob_gps_loss = 0.9; 
else
    % Robot is OUTSIDE the zone: Perfect or near-perfect reception
    prob_gps_loss = 0.0; % Or set to 0.05 if you want occasional random drops anywhere
end

if rnd < prob_gps_loss

     % ONLY ENCODERS 
    m = 2;
    
    y_measurement(1:2) = [
        measurements(4);
        measurements(5)
    ];

    H(1:2,:) = [
        0 0 0 1 0 0 0;
        0 0 0 0 1 0 0
    ];

    R = R_2;

    

else
            
        % FULL SENSING
        m = 5;
        
        % MoCap + ENCODERS + IMU 
        y_measurement(1:5) = [
            measurements(1) ;  % x
            measurements(2) ;  % y
            measurements(3) ;  % θ
            measurements(4);                   % Δφ_L
            measurements(5);                   % Δφ_R
        ];

        H(1:5,:) = [
            1 0 0 0 0 0 0;
            0 1 0 0 0 0 0;
            0 0 1 0 0 0 0;
            0 0 0 1 0 0 0;
            0 0 0 0 1 0 0;
           
        ];
      

        % Dynamically adjust measurement confidence based on the noise zone
        if index == 2
            % Inside the red zone: Sensors are noisy, trust the prediction more
            R = R_bad; 
        else
            % Outside the red zone: Sensors are clean, trust the measurements
            R = R_good; 
        end
        % R = R_5;


         
end


% Trim to actual sizes
y_measurement = y_measurement(1:m);
H = H(1:m, :);
R = R(1:m, 1:m);

err = y_measurement - H * z_pred;
S = H * P_pred * H' + R;
K = P_pred * H' / S;

% states update
z_KF_new = z_pred + K * err;

% covariance update
I = eye(size(P_pred));
P_KF_new = (I - K*H)*P_pred*(I - K*H)' + K*R*K';

% Normalize angle
z_KF_new(3) = atan2(sin(z_KF_new(3)), cos(z_KF_new(3)));

== matlab function online_robot_2024b/Odometry_IMU1 ==
  data: v input; q_est output; omega input; q_init input; Ts input
function q_est = fcn(v, omega, q_init, Ts)
    % Persistent variables hold their value between function calls
    persistent q_prev;
    
    if isempty(q_prev)
        q_prev = q_init;
    end
    
    % Dead-reckoning equations
    theta_new = q_prev(3) + omega * Ts;
    
    % Ensure angle is wrapped between -pi and pi
    theta_new = wrapToPi(theta_new);
    
    x_new = q_prev(1) + v * cos(theta_new) * Ts;
    y_new = q_prev(2) + v * sin(theta_new) * Ts;
    
    q_est = [x_new; y_new; theta_new];
    q_prev = q_est;
end

== matlab function online_robot_2024b/Controller ==
  data: q_est input; v output; q_target input; omega output; k1 input; k2 input; k3 input
function [v, omega] = fcn(q_est, q_target, k1, k2, k3)

    % Default outputs
    v = 0;
    omega = 0;
    
    % --- Internal Settings (instead of external constants) ---
    v_limit = 0.22;    % Maximum linear velocity [m/s]
    omega_limit = 10; % Maximum angular velocity according to project requirements [rad/s]
    
    % 1. Compute errors in polar coordinates
    dx = q_target(1) - q_est(1);
    dy = q_target(2) - q_est(2);
    
    rho = sqrt(dx^2 + dy^2);
    theta_target = atan2(dy, dx);
    
    gamma = wrapToPi(theta_target - q_est(3));
    delta = wrapToPi(gamma + q_est(3) - q_target(3));
    
    % 2. Control Law (Astolfi Controller)
    if rho < 0.05
        
        % Stop near the target
        v = 0;
        omega = 0;
        
    else
        
        % Compute linear velocity
        v = k1 * rho * cos(gamma);
        
        % Handle sinc(gamma) to avoid division by zero
        if abs(gamma) < 1e-4
            sinc_gamma = 1;
        else
            sinc_gamma = sin(gamma) / gamma;
        end
        
        % Compute angular velocity
        omega = k2 * gamma + ...
                k1 * sinc_gamma * cos(gamma) * (gamma + k3 * delta);
    end
    
    % 3. Apply saturation limits directly in the code
    if abs(v) > v_limit
        v = v_limit * sign(v);
    end
    
    if abs(omega) > omega_limit
        omega = omega_limit * sign(omega);
    end
end

== matlab function online_robot_2024b/Odometry_IMU ==
  data: v input; q_est output; omega input; q_init input; Ts input
function q_est = fcn_exact(v, omega, q_init, Ts)
    persistent q_prev;
    
    if isempty(q_prev)
        q_prev = q_init;
    end
    
    theta_prev = q_prev(3);
    theta_new = wrapToPi(theta_prev + omega * Ts);
    
    % Use a small tolerance to avoid division by zero when going straight
    if abs(omega) < 1e-6
        x_new = q_prev(1) + v * cos(theta_prev) * Ts;
        y_new = q_prev(2) + v * sin(theta_prev) * Ts;
    else
        x_new = q_prev(1) + (v / omega) * (sin(theta_prev + omega*Ts) - sin(theta_prev));
        y_new = q_prev(2) - (v / omega) * (cos(theta_prev + omega*Ts) - cos(theta_prev));
    end
    
    q_est = [x_new; y_new; theta_new];
    q_prev = q_est;
end

== matlab function online_robot_2024b/Fake_Vicon ==
  data: q_real input; Y_vicon_fake output
function Y_vicon_fake = fcn(q_real)

    % q_real is the odometry output,
    % assumed here to represent the robot's true position
    
    x = q_real(1);
    y = q_real(2);
    theta = q_real(3);
    
    % Simulate sensor noise inside the red zone
    % (between x = -0.6 and x = 0.2)
    if (x >= -0.6 && x <= 0.2)
        
        % Add Gaussian noise
        noise = 0.02 * randn(3,1);
        
        Y_vicon_fake = q_real + noise;
        
    else
        
        % Outside the red zone,
        % the sensor is assumed to be perfectly accurate
        Y_vicon_fake = q_real;
    end
end

== matlab function online_robot_2024b/Visualizer ==
  data: q_est input
function visualizer(q_est)
    coder.extrinsic('draw_robot');
    draw_robot(q_est(1), q_est(2));
end

== matlab function online_robot_2024b/Subsystem1/Subsystem/  ==
  data: y output; pos input; condition output
function [y, condition] = check(pos)

x1 = -2.9; y1 = -1.5;
x2 = -1.6; y2 = -1.1;
x3 = -1.5; y3 = -0.7;
x4 = -1.4; y4 = -0.3;
x5 = -0.6; y5 =  0.1;
x6 =  0.2; y6 =  1.5;
x7 =  1.0;
x8 =  1.1;
x9 =  2.9;

P_loss = 0.9;


if ((pos(1) >= x5) && (pos(1) <= x6)) && ((pos(2) >= y1) && (pos(2) <= y5))
    % add noise
    y = pos + 0.02*randn(3,1);
    condition = 1;
elseif ((pos(1) >= x7) && (pos(1) <= x9)) && ((pos(2) >= y1) && (pos(2) <= y6))
    % measurement loss
    if rand > P_loss
        y = pos;
    else
        y = 0*pos;
    end
    condition = 2;
else
    y = pos;
    condition = 0;
end
